simulink subsystem "Autonomous_Paths_and_Actions_sub"  (R2023b)
settings: Solver=VariableStepAuto  StartTime=0.0  StopTime=10.0  RelTol=1e-3
undefined symbols (not defined in the file): All_Paths_Num_Poses, All_Paths_Ref_Poses_Blue, All_Paths_Ref_Poses_Red, Spline_Max_Num_RefPoses, test_cases
settings Model: Creator=ander  LastModifiedBy=ander

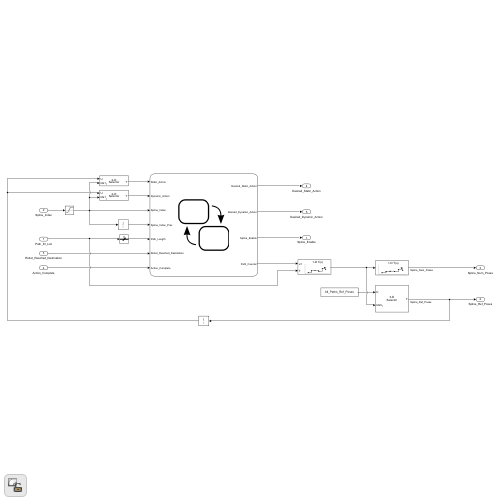
[thumbnail: Simulink's stored preview of the top-level diagram]
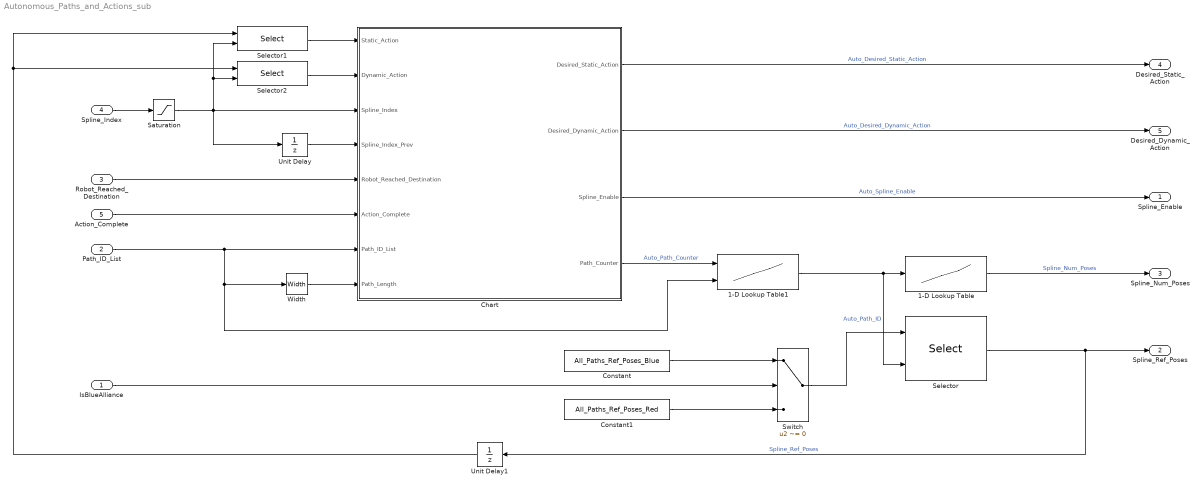
== system Autonomous_Paths_and_Actions_sub ==
  IsBlueAlliance : Inport
  Path_ID_List : Inport  Port=2
  Robot_Reached_Destination : Inport  Port=3
  Spline_Index : Inport  Port=4
  Action_Complete : Inport  Port=5
  1-D Lookup Table : Lookup_n-D  NumberOfTableDimensions=1  BreakpointsSpecification=Even spacing  BreakpointsForDimension1=[-5:5]  Table=All_Paths_Num_Poses  InterpMethod=Flat  InternalRulePriority=Speed  RndMeth=Simplest
  1-D Lookup Table1 : Lookup_n-D  NumberOfTableDimensions=1  BreakpointsSpecification=Even spacing  BreakpointsForDimension1=[-5:5]  TableSource=Input port  Table=test_cases  InterpMethod=Flat  InternalRulePriority=Speed  RndMeth=Simplest
      settings: InputPortMap=u0,p221
  Chart : Stateflow chart  TreatAsAtomicUnit=on
      settings: PortSchema="{\"entries\":[{\"content\":{\"sides\":[{\"content\":{\"connectorIds\":[\"In2\",\"In3\",\"In5\",\"In7\",\"In1\",\"In4\",\"In6\",\"In8\"]},\"type\":\"ConnectorPlacement.EquallySpacedRectSide\",\"uuid\":\"1968a818-e4ac-4b22-96eb-c360107c622f\"},{\"content\":{\"connectorIds\":[\"Out1\",\"Out2\",\"Out4\",\"Out3\"],\"side\":\"RIGHT\"},\"type\":\"ConnectorPlacement.EquallySpacedRectSide\",\"uuid\":\"7fe9b0f3-1e9a-4e98-a228-ddf13bcb20e0\"},{\"content\":{\"side\":\"TOP\"},\"type\":\"ConnectorPlacement.EquallySpacedRectSide\",\"uuid\":\"8ed6cee9-185e-462a-a993-54de90a47c55\"}]},\"type\":\"ConnectorPlacement.EquallySpacedConnector\",\"uuid\":\"6f1faf48-b95e-418c-8cdb-2f63138a33cf\"}],\"packageUris\":[\"http://schema.mathworks.com/mf0/Connector/R2020b\"],\"version\":\"1.0\"}"
  Constant : Constant  Value=All_Paths_Ref_Poses_Blue
  Constant1 : Constant  Value=All_Paths_Ref_Poses_Red
  Saturation : Saturate  UpperLimit=Spline_Max_Num_RefPoses  LowerLimit=1
  Selector : Selector  NumberOfDimensions=3  InputPortWidth=3  IndexOptions=Select all,Select all,Index vector (port)  Indices=[1 3],1,1  OutputSizes=1,1,1
  Selector1 : Selector  NumberOfDimensions=2  InputPortWidth=3  IndexOptions=Index vector (port),Index vector (dialog)  Indices=[1 3],[5]  OutputSizes=1,1
  Selector2 : Selector  NumberOfDimensions=2  InputPortWidth=3  IndexOptions=Index vector (port),Index vector (dialog)  Indices=[1 3],[6]  OutputSizes=1,1
  Switch : Switch  Criteria=u2 ~= 0  SaturateOnIntegerOverflow=off  InputSameDT=off
  Unit Delay : UnitDelay  SampleTime=-1  HasFrameUpgradeWarning=on
  Unit Delay1 : UnitDelay  SampleTime=-1  HasFrameUpgradeWarning=on
  Width : Width
  Spline_Enable : Outport
  Spline_Ref_Poses : Outport  Port=2
  Spline_Num_Poses : Outport  Port=3
  Desired_Static_Action : Outport  Port=4
  Desired_Dynamic_Action : Outport  Port=5
  wires:
  Path_ID_List/1 -> Chart/6(Path_ID_List), 1-D Lookup Table1/2, Width/1
  Width/1 -> Chart/8(Path_Length)
  Chart/4(Spline_Enable) -> Spline_Enable/1  "Auto_Spline_Enable"
  Unit Delay1/1 -> Selector1/1, Selector2/1
  1-D Lookup Table1/1 -> Selector/2, 1-D Lookup Table/1  "Auto_Path_ID"
  Chart/2(Desired_Dynamic_Action) -> Desired_Dynamic_Action/1  "Auto_Desired_Dynamic_Action"
  Saturation/1 -> Chart/5(Spline_Index), Selector1/2, Selector2/2, Unit Delay/1
  Spline_Index/1 -> Saturation/1
  1-D Lookup Table/1 -> Spline_Num_Poses/1  "Spline_Num_Poses"
  Chart/1(Desired_Static_Action) -> Desired_Static_Action/1  "Auto_Desired_Static_Action"
  Action_Complete/1 -> Chart/4(Action_Complete)
  Selector/1 -> Spline_Ref_Poses/1, Unit Delay1/1  "Spline_Ref_Poses"
  Selector1/1 -> Chart/2(Static_Action)
  Selector2/1 -> Chart/3(Dynamic_Action)
  Unit Delay/1 -> Chart/7(Spline_Index_Prev)
  Robot_Reached_Destination/1 -> Chart/1(Robot_Reached_Destination)
  Switch/1 -> Selector/1
  IsBlueAlliance/1 -> Switch/2
  Constant/1 -> Switch/1
  Constant1/1 -> Switch/3
  Chart/3(Path_Counter) -> 1-D Lookup Table1/1  "Auto_Path_Counter"

== stateflow chart Autonomous_Paths_and_Actions_sub/Chart ==
  state Start_Action
    entry: Spline_Enable = false;
    Desired_Static_Action = Static_Action;
    Desired_Dynamic_Action = 0;
    counter = 0;
    during:  Desired_Static_Action = Static_Action;
    counter = counter +1;
  state Follow_Path
    entry:
    Spline_Enable = true;
    Desired_Static_Action = 0;
    Desired_Dynamic_Action = Dynamic_Action;
  state End_Action
    entry:  Spline_Enable = false;
    Desired_Static_Action = Static_Action;
    Desired_Dynamic_Action = 0;
  (default) -> Start_Action : {Path_Counter = 1;}
  End_Action -> Start_Action : [(Desired_Static_Action == 0 || Action_Complete) && ...
      | Path_Counter < Path_Length && ...
      | Path_ID_List(Path_Counter + 1) ~= 0]
      | {Path_Counter = Path_Counter + 1;}
  Start_Action -> Follow_Path : [counter > 1 && (Desired_Static_Action == 0 || Action_Complete)]
  Follow_Path -> Follow_Path [order 2] : [Spline_Index > Spline_Index_Prev]
  Follow_Path -> End_Action [order 1] : [Robot_Reached_Destination]
  data: Robot_Reached_Destination input; Static_Action input; Dynamic_Action input; Action_Complete input; Spline_Index input; Path_ID_List input; Spline_Index_Prev input; Desired_Static_Action output; Desired_Dynamic_Action output; Path_Counter output; Path_Length input; Spline_Enable output boolean; counter local
